simulink model "mars_rover_terrain"  (R2025a)
settings: Solver=daessc  StartTime=0.0  StopTime=130*10  FixedStep=1e-10  MaxStep=1e-1  RelTol=1e-3  AbsTol=1e-3  EnableMultiTasking=on
undefined symbols (not defined in the file): arm_q0, Control, eeConfig, L1, L2, L3, LS1, LS3, R1, R2, R3, Rover, rover_path, RS1, RS3, X, Y, Z
libraries: sm_lib x137, nesl_utility x109, fl_lib x85, sdl_lib x20, ee_lib x10, mars_rover_lib x8, simulink x4, slpidlib x3, batteryecm_lib x2, robotcorelib x1, robotalgslib x1
(part 10 of 10)

== system mars_rover_terrain/Rover/Chassis/Powertrain/Electrical/Steer/Sense tR1 ==
  Ideal Torque Sensor : fl_lib/Mechanical/Mechanical Sensors/Ideal Torque Sensor
  PS-Simulink Converter6 : nesl_utility/PS-Simulink Converter  PhysicalDomain=network_engine_domain  SubClassName=ps_output  LeftPortType=input  RightPortType=output  PseudoPeriodic=off  Frequencies=[]  VectorFormat=1-D array  Unit=inherit  AffineConversion=off
  C : PMIOPort  Side=Right
  R : PMIOPort  Port=2  Side=Left
  T : Outport
  wires:
  PS-Simulink Converter6/1 -> T/1
  connections:
  Ideal Torque Sensor/RConn1 -- C/RConn1
  Ideal Torque Sensor/RConn2 -- PS-Simulink Converter6/LConn1
  Ideal Torque Sensor/LConn1 -- R/RConn1

== system mars_rover_terrain/Rover/Chassis/Powertrain/Electrical/Steer/Sense tR3 ==
  Ideal Torque Sensor : fl_lib/Mechanical/Mechanical Sensors/Ideal Torque Sensor
  PS-Simulink Converter6 : nesl_utility/PS-Simulink Converter  PhysicalDomain=network_engine_domain  SubClassName=ps_output  LeftPortType=input  RightPortType=output  PseudoPeriodic=off  Frequencies=[]  VectorFormat=1-D array  Unit=inherit  AffineConversion=off
  C : PMIOPort  Side=Right
  R : PMIOPort  Port=2  Side=Left
  T : Outport
  wires:
  PS-Simulink Converter6/1 -> T/1
  connections:
  Ideal Torque Sensor/RConn1 -- C/RConn1
  Ideal Torque Sensor/RConn2 -- PS-Simulink Converter6/LConn1
  Ideal Torque Sensor/LConn1 -- R/RConn1

== system mars_rover_terrain/Rover/Chassis/Powertrain/Electrical/Steer/Sensor iL1 ==
  Current Sensor : fl_lib/Electrical/Electrical Sensors/Current Sensor
  PS-Simulink Converter3 : nesl_utility/PS-Simulink Converter  PhysicalDomain=network_engine_domain  SubClassName=ps_output  LeftPortType=input  RightPortType=output  PseudoPeriodic=off  Frequencies=[]  VectorFormat=1-D array  Unit=inherit  AffineConversion=off
  + : PMIOPort  Side=Left
  - : PMIOPort  Port=2  Side=Right
  i : Outport
  wires:
  PS-Simulink Converter3/1 -> i/1
  connections:
  PS-Simulink Converter3/LConn1 -- Current Sensor/RConn1
  Current Sensor/RConn2 -- -/RConn1
  +/RConn1 -- Current Sensor/LConn1

== system mars_rover_terrain/Rover/Chassis/Powertrain/Electrical/Steer/Sensor iL3 ==
  Current Sensor : fl_lib/Electrical/Electrical Sensors/Current Sensor
  PS-Simulink Converter3 : nesl_utility/PS-Simulink Converter  PhysicalDomain=network_engine_domain  SubClassName=ps_output  LeftPortType=input  RightPortType=output  PseudoPeriodic=off  Frequencies=[]  VectorFormat=1-D array  Unit=inherit  AffineConversion=off
  + : PMIOPort  Side=Left
  - : PMIOPort  Port=2  Side=Right
  i : Outport
  wires:
  PS-Simulink Converter3/1 -> i/1
  connections:
  +/RConn1 -- Current Sensor/LConn1
  Current Sensor/RConn2 -- -/RConn1
  PS-Simulink Converter3/LConn1 -- Current Sensor/RConn1

== system mars_rover_terrain/Rover/Chassis/Powertrain/Electrical/Steer/Sensor iR1 ==
  Current Sensor : fl_lib/Electrical/Electrical Sensors/Current Sensor
  PS-Simulink Converter3 : nesl_utility/PS-Simulink Converter  PhysicalDomain=network_engine_domain  SubClassName=ps_output  LeftPortType=input  RightPortType=output  PseudoPeriodic=off  Frequencies=[]  VectorFormat=1-D array  Unit=inherit  AffineConversion=off
  + : PMIOPort  Side=Left
  - : PMIOPort  Port=2  Side=Right
  i : Outport
  wires:
  PS-Simulink Converter3/1 -> i/1
  connections:
  +/RConn1 -- Current Sensor/LConn1
  Current Sensor/RConn2 -- -/RConn1
  PS-Simulink Converter3/LConn1 -- Current Sensor/RConn1

== system mars_rover_terrain/Rover/Chassis/Powertrain/Electrical/Steer/Sensor iR3 ==
  Current Sensor : fl_lib/Electrical/Electrical Sensors/Current Sensor
  PS-Simulink Converter3 : nesl_utility/PS-Simulink Converter  PhysicalDomain=network_engine_domain  SubClassName=ps_output  LeftPortType=input  RightPortType=output  PseudoPeriodic=off  Frequencies=[]  VectorFormat=1-D array  Unit=inherit  AffineConversion=off
  + : PMIOPort  Side=Left
  - : PMIOPort  Port=2  Side=Right
  i : Outport
  wires:
  PS-Simulink Converter3/1 -> i/1
  connections:
  PS-Simulink Converter3/LConn1 -- Current Sensor/RConn1
  Current Sensor/RConn2 -- -/RConn1
  +/RConn1 -- Current Sensor/LConn1

== system mars_rover_terrain/Rover/Chassis/Powertrain/Ideal/Drive/Sense wL1 ==
  Ideal Rotational Motion Sensor : fl_lib/Mechanical/Mechanical Sensors/Ideal Rotational Motion Sensor  reference=foundation.enum.MeasurementReference.difference  acceleration_port=false  velocity_port=true  position_port=true  wrap_angle=simscape.enum.onoff.off  offset=0 rad
  PS Terminator : fl_lib/Physical Signals/Sinks/PS Terminator
  PS-Simulink Converter : nesl_utility/PS-Simulink Converter  PhysicalDomain=network_engine_domain  SubClassName=ps_output  LeftPortType=input  RightPortType=output  PseudoPeriodic=off  Frequencies=[]  VectorFormat=1-D array  Unit=inherit  AffineConversion=off
  R : PMIOPort  Side=Right
  C : PMIOPort  Port=2  Side=Left
  w : Outport
  wires:
  PS-Simulink Converter/1 -> w/1
  connections:
  Ideal Rotational Motion Sensor/RConn2 -- PS-Simulink Converter/LConn1
  Ideal Rotational Motion Sensor/LConn1 -- R/RConn1
  Ideal Rotational Motion Sensor/RConn1 -- C/RConn1
  Ideal Rotational Motion Sensor/RConn3 -- PS Terminator/LConn1

== system mars_rover_terrain/Rover/Chassis/Powertrain/Ideal/Drive/Sense wL2 ==
  Ideal Rotational Motion Sensor : fl_lib/Mechanical/Mechanical Sensors/Ideal Rotational Motion Sensor  reference=foundation.enum.MeasurementReference.difference  acceleration_port=false  velocity_port=true  position_port=true  wrap_angle=simscape.enum.onoff.off  offset=0 rad
  PS Terminator : fl_lib/Physical Signals/Sinks/PS Terminator
  PS-Simulink Converter : nesl_utility/PS-Simulink Converter  PhysicalDomain=network_engine_domain  SubClassName=ps_output  LeftPortType=input  RightPortType=output  PseudoPeriodic=off  Frequencies=[]  VectorFormat=1-D array  Unit=inherit  AffineConversion=off
  R : PMIOPort  Side=Right
  C : PMIOPort  Port=2  Side=Left
  w : Outport
  wires:
  PS-Simulink Converter/1 -> w/1
  connections:
  Ideal Rotational Motion Sensor/RConn3 -- PS Terminator/LConn1
  Ideal Rotational Motion Sensor/RConn1 -- C/RConn1
  Ideal Rotational Motion Sensor/LConn1 -- R/RConn1
  Ideal Rotational Motion Sensor/RConn2 -- PS-Simulink Converter/LConn1

== system mars_rover_terrain/Rover/Chassis/Powertrain/Ideal/Drive/Sense wL3 ==
  Ideal Rotational Motion Sensor : fl_lib/Mechanical/Mechanical Sensors/Ideal Rotational Motion Sensor  reference=foundation.enum.MeasurementReference.difference  acceleration_port=false  velocity_port=true  position_port=true  wrap_angle=simscape.enum.onoff.off  offset=0 rad
  PS Terminator : fl_lib/Physical Signals/Sinks/PS Terminator
  PS-Simulink Converter : nesl_utility/PS-Simulink Converter  PhysicalDomain=network_engine_domain  SubClassName=ps_output  LeftPortType=input  RightPortType=output  PseudoPeriodic=off  Frequencies=[]  VectorFormat=1-D array  Unit=inherit  AffineConversion=off
  R : PMIOPort  Side=Right
  C : PMIOPort  Port=2  Side=Left
  w : Outport
  wires:
  PS-Simulink Converter/1 -> w/1
  connections:
  Ideal Rotational Motion Sensor/RConn2 -- PS-Simulink Converter/LConn1
  Ideal Rotational Motion Sensor/LConn1 -- R/RConn1
  Ideal Rotational Motion Sensor/RConn1 -- C/RConn1
  Ideal Rotational Motion Sensor/RConn3 -- PS Terminator/LConn1

== system mars_rover_terrain/Rover/Chassis/Powertrain/Ideal/Drive/Sense wR1 ==
  Ideal Rotational Motion Sensor : fl_lib/Mechanical/Mechanical Sensors/Ideal Rotational Motion Sensor  reference=foundation.enum.MeasurementReference.difference  acceleration_port=false  velocity_port=true  position_port=true  wrap_angle=simscape.enum.onoff.off  offset=0 rad
  PS Terminator : fl_lib/Physical Signals/Sinks/PS Terminator
  PS-Simulink Converter : nesl_utility/PS-Simulink Converter  PhysicalDomain=network_engine_domain  SubClassName=ps_output  LeftPortType=input  RightPortType=output  PseudoPeriodic=off  Frequencies=[]  VectorFormat=1-D array  Unit=inherit  AffineConversion=off
  R : PMIOPort  Side=Right
  C : PMIOPort  Port=2  Side=Left
  w : Outport
  wires:
  PS-Simulink Converter/1 -> w/1
  connections:
  Ideal Rotational Motion Sensor/RConn2 -- PS-Simulink Converter/LConn1
  Ideal Rotational Motion Sensor/LConn1 -- R/RConn1
  Ideal Rotational Motion Sensor/RConn1 -- C/RConn1
  Ideal Rotational Motion Sensor/RConn3 -- PS Terminator/LConn1

== system mars_rover_terrain/Rover/Chassis/Powertrain/Ideal/Drive/Sense wR2 ==
  Ideal Rotational Motion Sensor : fl_lib/Mechanical/Mechanical Sensors/Ideal Rotational Motion Sensor  reference=foundation.enum.MeasurementReference.difference  acceleration_port=false  velocity_port=true  position_port=true  wrap_angle=simscape.enum.onoff.off  offset=0 rad
  PS Terminator : fl_lib/Physical Signals/Sinks/PS Terminator
  PS-Simulink Converter : nesl_utility/PS-Simulink Converter  PhysicalDomain=network_engine_domain  SubClassName=ps_output  LeftPortType=input  RightPortType=output  PseudoPeriodic=off  Frequencies=[]  VectorFormat=1-D array  Unit=inherit  AffineConversion=off
  R : PMIOPort  Side=Right
  C : PMIOPort  Port=2  Side=Left
  w : Outport
  wires:
  PS-Simulink Converter/1 -> w/1
  connections:
  Ideal Rotational Motion Sensor/RConn3 -- PS Terminator/LConn1
  Ideal Rotational Motion Sensor/RConn1 -- C/RConn1
  Ideal Rotational Motion Sensor/LConn1 -- R/RConn1
  Ideal Rotational Motion Sensor/RConn2 -- PS-Simulink Converter/LConn1

== system mars_rover_terrain/Rover/Chassis/Powertrain/Ideal/Drive/Sense wR3 ==
  Ideal Rotational Motion Sensor : fl_lib/Mechanical/Mechanical Sensors/Ideal Rotational Motion Sensor  reference=foundation.enum.MeasurementReference.difference  acceleration_port=false  velocity_port=true  position_port=true  wrap_angle=simscape.enum.onoff.off  offset=0 rad
  PS Terminator : fl_lib/Physical Signals/Sinks/PS Terminator
  PS-Simulink Converter : nesl_utility/PS-Simulink Converter  PhysicalDomain=network_engine_domain  SubClassName=ps_output  LeftPortType=input  RightPortType=output  PseudoPeriodic=off  Frequencies=[]  VectorFormat=1-D array  Unit=inherit  AffineConversion=off
  R : PMIOPort  Side=Right
  C : PMIOPort  Port=2  Side=Left
  w : Outport
  wires:
  PS-Simulink Converter/1 -> w/1
  connections:
  Ideal Rotational Motion Sensor/RConn2 -- PS-Simulink Converter/LConn1
  Ideal Rotational Motion Sensor/LConn1 -- R/RConn1
  Ideal Rotational Motion Sensor/RConn1 -- C/RConn1
  Ideal Rotational Motion Sensor/RConn3 -- PS Terminator/LConn1

== system mars_rover_terrain/Rover/Chassis/Powertrain/Ideal/Power/Sensing Temperature ==
  PS-Simulink Converter : nesl_utility/PS-Simulink Converter  PhysicalDomain=network_engine_domain  SubClassName=ps_output  LeftPortType=input  RightPortType=output  PseudoPeriodic=off  Frequencies=[]  VectorFormat=1-D array  Unit=inherit  AffineConversion=off
  Temperature Sensor : fl_lib/Thermal/Thermal Sensors/Temperature Sensor  temperature_measure=foundation.enum.MeasurementReference.difference
  Thermal Reference : fl_lib/Thermal/Thermal Elements/Thermal Reference
  A : PMIOPort  Side=Left
  T : Outport
  wires:
  PS-Simulink Converter/1 -> T/1
  connections:
  Thermal Reference/LConn1 -- Temperature Sensor/RConn1
  Temperature Sensor/RConn2 -- PS-Simulink Converter/LConn1
  A/RConn1 -- Temperature Sensor/LConn1

== system mars_rover_terrain/Rover/Chassis/Powertrain/Ideal/Steer/Sense wL1 ==
  Ideal Rotational Motion Sensor : fl_lib/Mechanical/Mechanical Sensors/Ideal Rotational Motion Sensor  reference=foundation.enum.MeasurementReference.difference  acceleration_port=false  velocity_port=true  position_port=true  wrap_angle=simscape.enum.onoff.off  offset=0 rad
  PS Terminator : fl_lib/Physical Signals/Sinks/PS Terminator
  PS-Simulink Converter : nesl_utility/PS-Simulink Converter  PhysicalDomain=network_engine_domain  SubClassName=ps_output  LeftPortType=input  RightPortType=output  PseudoPeriodic=off  Frequencies=[]  VectorFormat=1-D array  Unit=inherit  AffineConversion=off
  R : PMIOPort  Side=Right
  C : PMIOPort  Port=2  Side=Left
  w : Outport
  wires:
  PS-Simulink Converter/1 -> w/1
  connections:
  Ideal Rotational Motion Sensor/RConn2 -- PS-Simulink Converter/LConn1
  Ideal Rotational Motion Sensor/LConn1 -- R/RConn1
  Ideal Rotational Motion Sensor/RConn1 -- C/RConn1
  Ideal Rotational Motion Sensor/RConn3 -- PS Terminator/LConn1

== system mars_rover_terrain/Rover/Chassis/Powertrain/Ideal/Steer/Sense wL3 ==
  Ideal Rotational Motion Sensor : fl_lib/Mechanical/Mechanical Sensors/Ideal Rotational Motion Sensor  reference=foundation.enum.MeasurementReference.difference  acceleration_port=false  velocity_port=true  position_port=true  wrap_angle=simscape.enum.onoff.off  offset=0 rad
  PS Terminator : fl_lib/Physical Signals/Sinks/PS Terminator
  PS-Simulink Converter : nesl_utility/PS-Simulink Converter  PhysicalDomain=network_engine_domain  SubClassName=ps_output  LeftPortType=input  RightPortType=output  PseudoPeriodic=off  Frequencies=[]  VectorFormat=1-D array  Unit=inherit  AffineConversion=off
  R : PMIOPort  Side=Right
  C : PMIOPort  Port=2  Side=Left
  w : Outport
  wires:
  PS-Simulink Converter/1 -> w/1
  connections:
  Ideal Rotational Motion Sensor/RConn2 -- PS-Simulink Converter/LConn1
  Ideal Rotational Motion Sensor/LConn1 -- R/RConn1
  Ideal Rotational Motion Sensor/RConn1 -- C/RConn1
  Ideal Rotational Motion Sensor/RConn3 -- PS Terminator/LConn1

== system mars_rover_terrain/Rover/Chassis/Powertrain/Ideal/Steer/Sense wR1 ==
  Ideal Rotational Motion Sensor : fl_lib/Mechanical/Mechanical Sensors/Ideal Rotational Motion Sensor  reference=foundation.enum.MeasurementReference.difference  acceleration_port=false  velocity_port=true  position_port=true  wrap_angle=simscape.enum.onoff.off  offset=0 rad
  PS Terminator : fl_lib/Physical Signals/Sinks/PS Terminator
  PS-Simulink Converter : nesl_utility/PS-Simulink Converter  PhysicalDomain=network_engine_domain  SubClassName=ps_output  LeftPortType=input  RightPortType=output  PseudoPeriodic=off  Frequencies=[]  VectorFormat=1-D array  Unit=inherit  AffineConversion=off
  R : PMIOPort  Side=Right
  C : PMIOPort  Port=2  Side=Left
  w : Outport
  wires:
  PS-Simulink Converter/1 -> w/1
  connections:
  Ideal Rotational Motion Sensor/RConn2 -- PS-Simulink Converter/LConn1
  Ideal Rotational Motion Sensor/LConn1 -- R/RConn1
  Ideal Rotational Motion Sensor/RConn1 -- C/RConn1
  Ideal Rotational Motion Sensor/RConn3 -- PS Terminator/LConn1

== system mars_rover_terrain/Rover/Chassis/Powertrain/Ideal/Steer/Sense wR3 ==
  Ideal Rotational Motion Sensor : fl_lib/Mechanical/Mechanical Sensors/Ideal Rotational Motion Sensor  reference=foundation.enum.MeasurementReference.difference  acceleration_port=false  velocity_port=true  position_port=true  wrap_angle=simscape.enum.onoff.off  offset=0 rad
  PS Terminator : fl_lib/Physical Signals/Sinks/PS Terminator
  PS-Simulink Converter : nesl_utility/PS-Simulink Converter  PhysicalDomain=network_engine_domain  SubClassName=ps_output  LeftPortType=input  RightPortType=output  PseudoPeriodic=off  Frequencies=[]  VectorFormat=1-D array  Unit=inherit  AffineConversion=off
  R : PMIOPort  Side=Right
  C : PMIOPort  Port=2  Side=Left
  w : Outport
  wires:
  PS-Simulink Converter/1 -> w/1
  connections:
  Ideal Rotational Motion Sensor/RConn2 -- PS-Simulink Converter/LConn1
  Ideal Rotational Motion Sensor/LConn1 -- R/RConn1
  Ideal Rotational Motion Sensor/RConn1 -- C/RConn1
  Ideal Rotational Motion Sensor/RConn3 -- PS Terminator/LConn1

== matlab function mars_rover_terrain/Control/Arm Control/ Trajectory Planner/Planner Subsystem/Inverse Kinematics ==
  data: jointSpaceWayPts output; eePoseDes input; eeIgs input; samplePosition input; prevWayPts input
function  jointSpaceWayPts = fcn(eePoseDes,eeIgs,samplePosition,prevWayPts)
% Wrapper around sm_mars_rover_arm_ik.m
% Takes end effector targets and initial guesses and returns all the
% actuator positions corresponding to each target.

coder.extrinsic("sm_mars_rover_arm_ik");

jointSpaceWayPts = zeros(7,6); %#ok<PREALL>

% Overwrite end effector target positions for
% acquiring sample with measurement from chassis
eePoseDes(3,1:3) = samplePosition + [0 0 0.1]; % Approach example from above
eePoseDes(4,1:3) = samplePosition;

% Obtain joint space waypoints by calling IK for each end effector target
if prevWayPts == zeros(7,6)
    [jointSpaceWayPts,solvedFlag] =  sm_mars_rover_arm_ik(eePoseDes,eeIgs); %#ok<ASGLU>
else
    jointSpaceWayPts = prevWayPts;
end

end

== matlab function mars_rover_terrain/Control/Chassis Control/Target Dir To Bicycle Steer Angle/Rad2Deg ==
  data: u input; y output
function y = fcn(u)
y = rad2deg(u);

== matlab function mars_rover_terrain/Rover/Chassis DOF/theta_act ==
  data: u input; z output; y output; x output
function [z,y,x] = fcn(u)
out = quat2eul(u');
z = out(1);
y = out(2);
x = out(3);
end

== matlab function mars_rover_terrain/Control/Chassis Control/Target Direction and Speed/Trapezoidal Vel Profile ==
  data: t input; startTime input; accel input; deaccelStartTime input; linVel input; lin_Vel_out output
function lin_Vel_out = fcn(t,startTime,accel,deaccelStartTime,linVel)
% Function to create a trapezoidal profile for rover's desired linear
% velocity

t2 = linVel/accel + startTime;
t3 = deaccelStartTime + 0.2;
tf = linVel/accel + t3;

if t>=startTime && t<t2 
    lin_Vel_out = accel*(t-startTime);

elseif t>=t2 && t < t3 
    lin_Vel_out = linVel;

elseif t>= t3 && t < tf 
    lin_Vel_out = linVel-accel*(t-t3);

else
    lin_Vel_out = 0;    
end


end

== matlab function mars_rover_terrain/Control/Chassis Control/Ackerman Steer Angle/Ackerman Steering Angle Formulation ==
  data: delta input; qSteerL3 output; L input; qSteerR3 output; d input; R output; L_R output; R_R output
function [qSteerL3,qSteerR3,R,L_R,R_R] = fcn(delta,L,d)
% Function to compute ackerman steering angles 
% from a bicycle steer angle.

R = L/tand(abs(delta));

if delta < 0
    qSteerL3 = atan2d(L,(R+d/2));
    qSteerR3 = atan2d(L,(R-d/2));
    L_R = (R+d/2);
    R_R = (R-d/2);
else
    qSteerL3 = -atan2d(L,(R-d/2));
    qSteerR3 = -atan2d(L,(R+d/2));
    L_R = (R-d/2);
    R_R = (R+d/2);
end

end

== matlab function mars_rover_terrain/Control/Chassis Control/Chassis Velocity To Wheel Speed ==
  data: vTarget input; steer_ang input; A3_ROC input; L3_ROC input; R3_ROC input; wL1 output; wheel_r input; wL2 output; wL3 output; L input; wR1 output; wR2 output; wR3 output
function [wL1,wL2,wL3, wR1,wR2,wR3] = ...
    fcn(vTarget,steer_ang,A3_ROC,L3_ROC,R3_ROC,wheel_r,L)
% Function to compute wheel speed from a desired linear velocity and
% desired path.

if any(abs(steer_ang) > 0)

    wL1 = (vTarget/wheel_r)*sqrt(L3_ROC^2 + L^2)/A3_ROC;
    wL2 = vTarget * L3_ROC/(A3_ROC*wheel_r);
    wL3 = (vTarget/wheel_r)*sqrt(L3_ROC^2 + L^2)/A3_ROC;
    wR1 = (vTarget/wheel_r)*sqrt(R3_ROC^2 + L^2)/A3_ROC;
    wR2 = vTarget * R3_ROC/(A3_ROC*wheel_r);
    wR3 = (vTarget/wheel_r)*sqrt(R3_ROC^2 + L^2)/A3_ROC;

else
    wL1 = vTarget / wheel_r;
    wL2 = vTarget / wheel_r;
    wL3 = vTarget / wheel_r;
    wR1 = vTarget / wheel_r;
    wR2 = vTarget / wheel_r;
    wR3 = vTarget / wheel_r;
end

end

== matlab function mars_rover_terrain/Control/Arm Control/ Trajectory Planner/Planner Subsystem/Task Scheduler ==
  settings: updateMethod=DISCRETE
  data: wayPts output; reset_t output; samplePickCmd output; sampleDropCmd output; actJointAngles input; desJointAngles input; samplePickSense input; sampleDropSense input; currentTime input; roverModePrev input; roverMode output
function [wayPts,reset_t,samplePickCmd,sampleDropCmd,roverMode]  = fcn(actJointAngles,desJointAngles,samplePickSense,sampleDropSense,currentTime,roverModePrev)
% This function plans the top level tasks for the arm. The end effector goal
% and sample interaction joint configuration modes depend on the current task mode.
%
% mode 0: home/initial position (waypt 1) (samplePickCmd Off)
% mode 1-2: move to the position close the sample (waypt 3 via waypt 2) (samplePickCmd Off)
% mode 3-4 : move to sample position and pick up sample (waypt 4) (samplePickCmd On)
% mode 5 : move back to the position close the sample (waypt 3) (samplePickCmd On)
% mode 6 : move to the position close to the sample storage unit (waypt 5) (samplePickCmd On)
% mode 7-8 : move to sample storage position and drop/collect sample (waypt 6) (sampleDropCmd On)
% mode 9 : move back to the position close to the sample storage unit (samplePickCmd,sampleDropCmd On)
% mode 10-11 :move to home position

maxErrPos = 0.5;
actJointAngles =actJointAngles';
persistent resetTime

roverMode = roverModePrev;

if isempty(resetTime)
    %roverMode = 0;
    resetTime = 0;
end

reset_t =  resetTime;

switch roverMode

    case 0
        % Home Position
        wayPts = [desJointAngles(1,:);desJointAngles(1,:)];
        samplePickCmd = false;
        sampleDropCmd = false;

        if all(abs(actJointAngles-desJointAngles(1,:)) < maxErrPos)
            resetTime = currentTime;
            if sampleDropSense == 1
                roverMode = 0;
            else
                roverMode = 1;
            end
        end

    case 1

        wayPts = desJointAngles(1:2,:);
        samplePickCmd = false;
        sampleDropCmd = false;

        if all(abs(actJointAngles-desJointAngles(2,:)) < maxErrPos)
            resetTime = currentTime;
            roverMode = 2;
        end

    case 2
        % Move to the position close the sample
        wayPts = desJointAngles(2:3,:);
        samplePickCmd = false;
        sampleDropCmd = false;

        if all(abs(actJointAngles-desJointAngles(3,:)) < maxErrPos)
            resetTime = currentTime;
            roverMode = 3;
        end

    case 3
        % Move to sample position
        wayPts = desJointAngles(3:4,:);
        samplePickCmd = false;
        sampleDropCmd = false;

        if all(abs(actJointAngles-desJointAngles(4,:)) < maxErrPos)
            resetTime = currentTime;
            roverMode = 4;
        end

    case 4
        % Stay at sample position and pick up the sample
        wayPts = [desJointAngles(4,:); desJointAngles(4,:)];
        samplePickCmd = true;
        sampleDropCmd = false;

        if all(abs(actJointAngles-desJointAngles(4,:)) < maxErrPos) && samplePickSense == 1
            resetTime = currentTime;
            roverMode = 5;
        end

    case 5
        % Move back to the position close to the sample
        wayPts = desJointAngles(4:-1:3,:);
        samplePickCmd = true;
        sampleDropCmd = false;

        if all(abs(actJointAngles-desJointAngles(3,:)) < maxErrPos)
            resetTime = currentTime;
            roverMode = 6;
        end


    case 6
        % Move the position close to the sample storage unit
        wayPts = [desJointAngles(3,:) ;desJointAngles(5,:)];
        samplePickCmd = true;
        sampleDropCmd = false;

        if all(abs(actJointAngles-desJointAngles(5,:)) < maxErrPos)
            resetTime = currentTime;
            roverMode = 7;
        end

    case 7
        % Move to the sample storage unit position
        wayPts = desJointAngles(5:6,:);
        sampleDropCmd = false;
        samplePickCmd = true;

        if all(abs(actJointAngles-desJointAngles(6,:)) < maxErrPos)
            resetTime = currentTime;
            roverMode = 8;
        end

    case 8
        % Stay at sample drop position, drop and collect the sample
        wayPts = [desJointAngles(6,:);desJointAngles(6,:)];

        sampleDropCmd = true;
        samplePickCmd = true;

        if (all(abs(actJointAngles-desJointAngles(6,:)) < maxErrPos)) && sampleDropSense == 1
            resetTime = currentTime;
            roverMode = 9;
        end

    case 9
        % Move back to the position close to the sample storage unit
        wayPts = desJointAngles(6:-1:5,:);
        sampleDropCmd = true;
        samplePickCmd = true;

        if all(abs(actJointAngles-desJointAngles(5,:)) < maxErrPos)
            resetTime = currentTime;
            roverMode = 10;
        end

    case 10
        % Move to home position via waypt 2
        wayPts = [desJointAngles(5,:); desJointAngles(7,:)];
        sampleDropCmd = true;
        samplePickCmd = true;

        if all(abs(actJointAngles-desJointAngles(7,:)) < maxErrPos)
            resetTime = currentTime;
            roverMode = 11;
        end

    case 11
        % Move to home position
        wayPts = [desJointAngles(7,:); desJointAngles(1,:)];
        sampleDropCmd = true;
        samplePickCmd = true;

        if all(abs(actJointAngles-desJointAngles(1,:)) < maxErrPos)
            resetTime = currentTime;
            roverMode = 12;
        end

    case 12
        % Mission Complete
        wayPts = [desJointAngles(7,:); desJointAngles(1,:)];
        sampleDropCmd = true;
        samplePickCmd = true;
        roverMode = 12;

    otherwise
        wayPts = [desJointAngles(1,:);desJointAngles(1,:)];
        samplePickCmd = false;
        sampleDropCmd = false;
        error('invalid mode');

end

end
